simulink model "lazo_orientacion"  (R2026a)
settings: Solver=ode1  StopTime=PL.t_fin  FixedStep=1e-3
values from neighbouring files (symbols this model uses):
  K = V_dis/PT.ke    [parametros_traccion.m]    (also in simular_escenarios.m = KE; K.umbral = u; simular_traccion.m = KT; K.cuentas = P.cuentas)
undefined symbols (not defined in the file or in its folder): PL
settings Model: Creator=Mitsuki  LastModifiedBy=Mitsuki

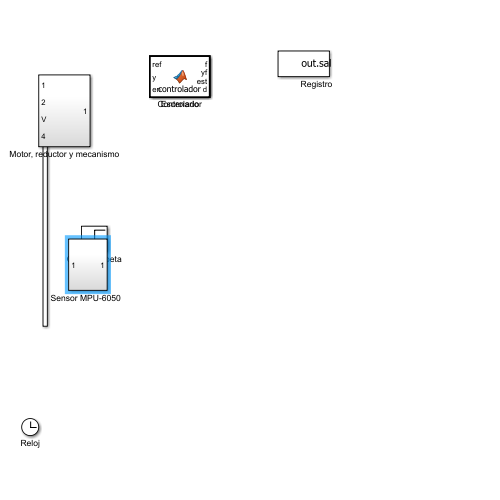
[thumbnail: Simulink's stored preview of the top-level diagram]
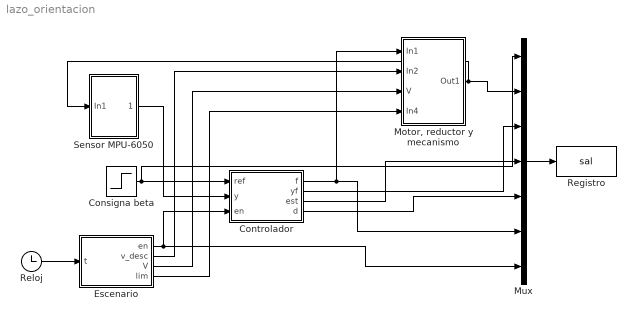
== system lazo_orientacion ==
  Consigna beta : Step  Time=PL.t_ref  InitialValue=PL.b_ini  FinalValue=PL.b_fin  SampleTime=0
  Controlador : MATLAB Function  TreatAsAtomicUnit=on
  Escenario : MATLAB Function  TreatAsAtomicUnit=on
  "Motor, reductor y mecanismo" : Subsystem
  Mux : Mux  Inputs=7
  Registro : ToWorkspace  VariableName=sal  SampleTime=K.Ts
  Reloj : Clock
  Sensor MPU-6050 : Subsystem
  wires:
  Consigna beta/1 -> Mux/1, Controlador/1(ref)
  Reloj/1 -> Escenario/1(t)
  Escenario/3(V) -> "Motor, reductor y mecanismo"/3(V)
  Controlador/4(d) -> Mux/5
  Sensor MPU-6050/1(Out1) -> Controlador/2(y)
  Escenario/4(lim) -> "Motor, reductor y mecanismo"/4(In4)
  Escenario/1(en) -> Mux/7, Controlador/3(en)
  Escenario/2(v_desc) -> "Motor, reductor y mecanismo"/2(In2)
  Controlador/1(f) -> Mux/6, "Motor, reductor y mecanismo"/1(In1)
  Controlador/2(yf) -> Mux/3
  Controlador/3(est) -> Mux/4
  "Motor, reductor y mecanismo"/1(Out1) -> Sensor MPU-6050/1(In1), Mux/2
  Mux/1 -> Registro/1

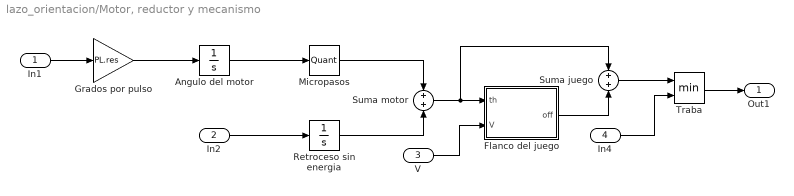
== system lazo_orientacion/Motor, reductor y mecanismo ==
  In1 : Inport
  In2 : Inport  Port=2
  V : Inport  Port=3
  In4 : Inport  Port=4
  Angulo del motor : Integrator  InitialCondition=PL.th0
  Flanco del juego : MATLAB Function  TreatAsAtomicUnit=on
  Grados por pulso : Gain  Gain=PL.res
  Micropasos : Quantizer  QuantizationInterval=PL.res
  Retroceso sin energia : Integrator
  Suma juego : Sum
  Suma motor : Sum
  Traba : MinMax  Inputs=2
  Out1 : Outport
  wires:
  Retroceso sin energia/1 -> Suma motor/2
  In2/1 -> Retroceso sin energia/1
  In1/1 -> Grados por pulso/1
  Grados por pulso/1 -> Angulo del motor/1
  Angulo del motor/1 -> Micropasos/1
  Micropasos/1 -> Suma motor/1
  Suma motor/1 -> Suma juego/1, Flanco del juego/1(th)
  V/1 -> Flanco del juego/2(V)
  Flanco del juego/1(off) -> Suma juego/2
  Suma juego/1 -> Traba/1
  In4/1 -> Traba/2
  Traba/1 -> Out1/1

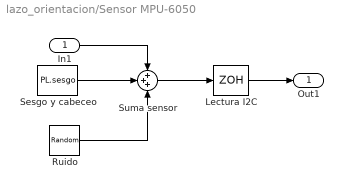
== system lazo_orientacion/Sensor MPU-6050 ==
  In1 : Inport
  Lectura I2C : ZeroOrderHold  SampleTime=K.Ts
  Ruido : RandomNumber  Variance=PL.sigma^2  Seed=PL.semilla  SampleTime=K.Ts
  Sesgo y cabeceo : Constant  Value=PL.sesgo
  Suma sensor : Sum  Inputs=+++
  Out1 : Outport
  wires:
  In1/1 -> Suma sensor/1
  Sesgo y cabeceo/1 -> Suma sensor/2
  Lectura I2C/1 -> Out1/1
  Ruido/1 -> Suma sensor/3
  Suma sensor/1 -> Lectura I2C/1

== matlab function lazo_orientacion/Controlador ==
  settings: updateMethod=DISCRETE  sampleTime=K.Ts
  data: ref input; f output; y input; en input; yf output; est output; d output; K parameter
function [f, yf, est, d] = controlador(ref, y, en, K)
% Lazo de posición del Arduino (ejecuta cada K.Ts).
%   ref  consigna de ángulo [grados]      y   lectura del MPU-6050 [grados]
%   en   1 con energía, 0 en parada        f   pulsos/s hacia el driver DM542
%   yf   lectura filtrada                  est 1 medir, 2 mover, 3 en banda, 4 falla
%   d    discrepancia pasos comandados - giro medido [grados]
persistent st yfs pc v cmdf cmdf0 yf0 tgt t_esp ref_ant ini
if isempty(st)
    st = 1; yfs = y; pc = y; v = 0; cmdf = y; cmdf0 = y; yf0 = y;
    tgt = y; t_esp = 0; ref_ant = ref; ini = false;
end
d = 0;
if en < 0.5
    % Parada: el Arduino queda sin energía; al rearmar arranca desde cero
    ini = false; st = 1; v = 0; f = 0; yf = y; est = 0;
    return
end
if ~ini
    yfs = y; pc = y; cmdf = y; v = 0; st = 1; t_esp = 0; ini = true;
end
yfs = yfs + K.a*(y - yfs);
r = min(max(ref, K.lim_min), K.lim_max);
if abs(r - ref_ant) > 1e-9 && st ~= 4
    if st == 3
        t_esp = K.T_asent;   % en reposo el filtro ya está asentado
    else
        t_esp = 0;
    end
    st = 1;
end
ref_ant = r;
switch st
    case 1  % medir: espera a que se asiente el filtro
        v = 0;
        t_esp = t_esp + K.Ts;
        if t_esp >= K.T_asent
            e = r - yfs;
            if abs(e) <= K.banda
                st = 3;
            else
                if K.dir_final ~= 0 && sign(e) ~= K.dir_final
                    D = K.Kp*e - K.dir_final*K.a_off;   % pasa la consigna y vuelve en el sentido final
                else
                    D = K.Kp*e;
                end
                tgt = pc + D; cmdf0 = cmdf; yf0 = yfs; st = 2;
            end
        end
    case 2  % mover con perfil trapezoidal
        dr = tgt - pc;
        vm = min([K.wmax, sqrt(2*K.alfa*abs(dr)), abs(v) + K.alfa*K.Ts]);
        if abs(dr) <= vm*K.Ts
            v = dr/K.Ts; st = 1; t_esp = 0;
        else
            v = sign(dr)*vm;
        end
        d = (cmdf - cmdf0) - (yfs - yf0);
        if abs(d) > K.umbral
            v = 0; st = 4;
        end
        if (yfs > K.lim_max + K.banda && v > 0) || (yfs < K.lim_min - K.banda && v < 0)
            v = 0; st = 4;
        end
    case 3  % en banda: vigila la deriva
        v = 0;
        if abs(r - yfs) > K.banda_re
            st = 1; t_esp = 0;   % espera a que el filtro se asiente antes de corregir
        end
    otherwise  % falla: motor detenido
        v = 0;
end
pc = pc + v*K.Ts;
cmdf = cmdf + K.a*(pc - cmdf);
f = v/K.res;
yf = yfs;
est = st;

== matlab function lazo_orientacion/Escenario ==
  data: t input; en output; v_desc output; V output; lim output; PL parameter
function [en, v_desc, V, lim] = escenario(t, PL)
en = 1; v_desc = 0; lim = 1e3;
V = 0;
if t >= PL.t_rafaga(1) && t < PL.t_rafaga(2), V = PL.V_rafaga; end

== matlab function lazo_orientacion/Motor, reductor y mecanismo/Flanco del juego ==
  data: th input; off output; V input; PL parameter
function off = flanco(th, V, PL)
% Momento de retención del peso del sensor y la placa (MC-15) menos la ráfaga,
% que actúa en sentido opuesto. Si cambia de signo, la corona cruza el juego.
M = PL.Kret*sind(th) - sign(th)*PL.Kv*V^2;
off = PL.b2*sign(M);
